simulink model "remus100_esekf_integrated"  (R2026b)
settings: Solver=ode4  StopTime=2668  FixedStep=0.01
InitFcn:
  | init_remus100_esekf_simulink;
values from neighbouring files (symbols this model uses):
  betaVc = deg2rad(150)    [init_remus100_esekf_simulink.m]    (also in run_fossen_esekf_integrated.m; run_fossen_standalone.m; sfun_remus100_plant.m = block.InputPort(3).Data)
  Vc = 0.5    [init_remus100_esekf_simulink.m]    (also in run_fossen_esekf_integrated.m; run_fossen_standalone.m; sfun_remus100_plant.m = block.InputPort(2).Data)
settings Model: Creator=Thinkpad  LastModifiedBy=Thinkpad

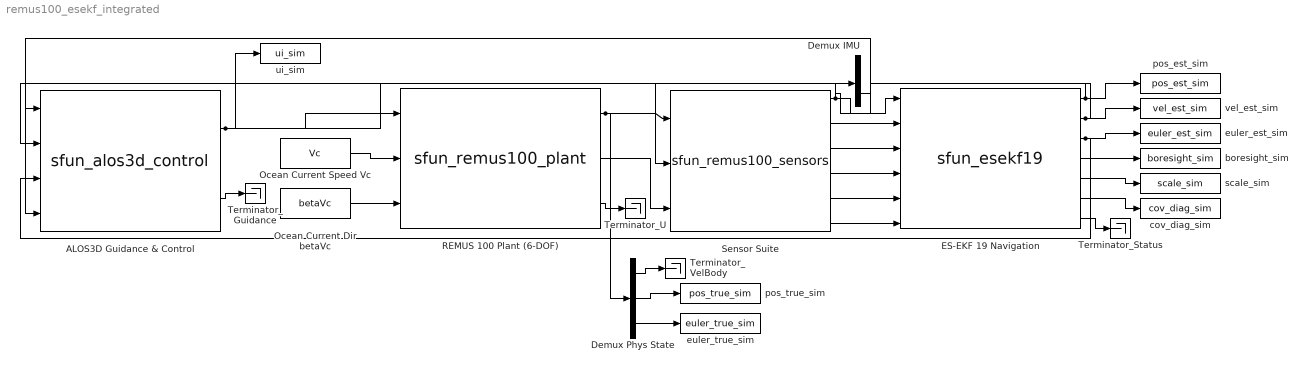
== system remus100_esekf_integrated ==
  ALOS3D Guidance & Control : M-S-Function  FunctionName=sfun_alos3d_control  Parameters=wpt, ctrl_prm
  Demux IMU : Demux  Outputs=[3 3]
  Demux Phys State : Demux  Outputs=[6 3 3]
  ES-EKF 19 Navigation : M-S-Function  FunctionName=sfun_esekf19  Parameters=cfg, noise_cfg
  Ocean Current Dir betaVc : Constant  Value=betaVc
  Ocean Current Speed Vc : Constant  Value=Vc
  REMUS 100 Plant (6-DOF) : M-S-Function  FunctionName=sfun_remus100_plant  Parameters=x0, 0.1
  Sensor Suite : M-S-Function  FunctionName=sfun_remus100_sensors  Parameters=sensor_params
  Terminator_Guidance : Terminator
  Terminator_Status : Terminator
  Terminator_U : Terminator
  Terminator_VelBody : Terminator
  boresight_sim : ToWorkspace  VariableName=boresight_sim  SampleTime=0.01
  cov_diag_sim : ToWorkspace  VariableName=cov_diag_sim  SampleTime=0.01
  euler_est_sim : ToWorkspace  VariableName=euler_est_sim  SampleTime=0.01
  euler_true_sim : ToWorkspace  VariableName=euler_true_sim  SampleTime=0.01
  pos_est_sim : ToWorkspace  VariableName=pos_est_sim  SampleTime=0.01
  pos_true_sim : ToWorkspace  VariableName=pos_true_sim  SampleTime=0.01
  scale_sim : ToWorkspace  VariableName=scale_sim  SampleTime=0.01
  ui_sim : ToWorkspace  VariableName=ui_sim  SampleTime=0.01
  vel_est_sim : ToWorkspace  VariableName=vel_est_sim  SampleTime=0.01
  wires:
  ALOS3D Guidance & Control/1 -> REMUS 100 Plant (6-DOF)/1, Sensor Suite/2, ui_sim/1
  ALOS3D Guidance & Control/2 -> Terminator_Guidance/1
  Ocean Current Speed Vc/1 -> REMUS 100 Plant (6-DOF)/2
  Ocean Current Dir betaVc/1 -> REMUS 100 Plant (6-DOF)/3
  REMUS 100 Plant (6-DOF)/1 -> Sensor Suite/1, Demux Phys State/1
  REMUS 100 Plant (6-DOF)/2 -> Sensor Suite/3
  REMUS 100 Plant (6-DOF)/3 -> Terminator_U/1
  Demux Phys State/1 -> Terminator_VelBody/1
  Demux Phys State/2 -> pos_true_sim/1
  Demux Phys State/3 -> euler_true_sim/1
  Sensor Suite/1 -> ES-EKF 19 Navigation/1, Demux IMU/1
  Sensor Suite/2 -> ES-EKF 19 Navigation/2
  Sensor Suite/3 -> ES-EKF 19 Navigation/3
  Sensor Suite/4 -> ES-EKF 19 Navigation/4
  Sensor Suite/5 -> ES-EKF 19 Navigation/5
  Sensor Suite/6 -> ES-EKF 19 Navigation/6
  Demux IMU/2 -> ALOS3D Guidance & Control/4
  ES-EKF 19 Navigation/1 -> ALOS3D Guidance & Control/1, pos_est_sim/1
  ES-EKF 19 Navigation/2 -> ALOS3D Guidance & Control/2, vel_est_sim/1
  ES-EKF 19 Navigation/3 -> ALOS3D Guidance & Control/3, euler_est_sim/1
  ES-EKF 19 Navigation/4 -> boresight_sim/1
  ES-EKF 19 Navigation/5 -> scale_sim/1
  ES-EKF 19 Navigation/6 -> cov_diag_sim/1
  ES-EKF 19 Navigation/7 -> Terminator_Status/1
